simulink model "HA_sim"  (R2023b)
settings: Solver=VariableStepAuto  StartTime=0.0  StopTime=10.0  RelTol=1e-3
InitFcn:
  | HA_Parameters;
values from neighbouring files (symbols this model uses):
  g = 9.81    [HA_Parameters.m]
  J = 10.4    [HA_Parameters.m]
  l = 1.5    [HA_Parameters.m]
  L = 2    [HA_Parameters.m]
  m = 5    [HA_Parameters.m]
  M = 75    [HA_Parameters.m]
libraries: vrlib x5
settings Model: Creator=vcichella  LastModifiedBy=vcichella
settings ModelReferenceCC: EnableRefExpFcnMdlSchedulingChecks=on

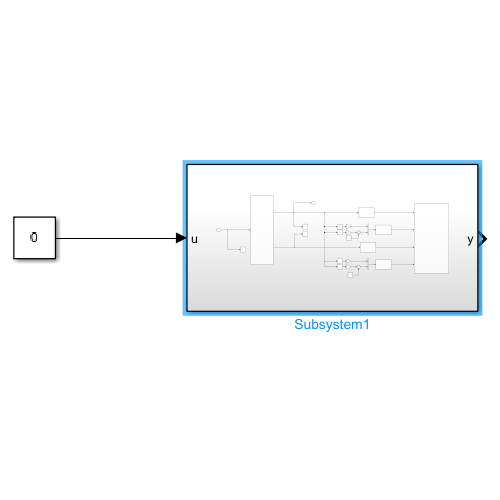
[thumbnail: Simulink's stored preview of the top-level diagram]
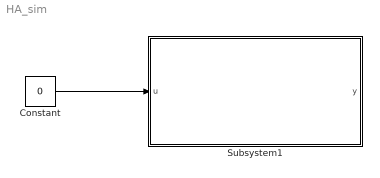
== system HA_sim ==
  Constant : Constant  Value=0
  Subsystem1 : Subsystem
  wires:
  Constant/1 -> Subsystem1/1(u)

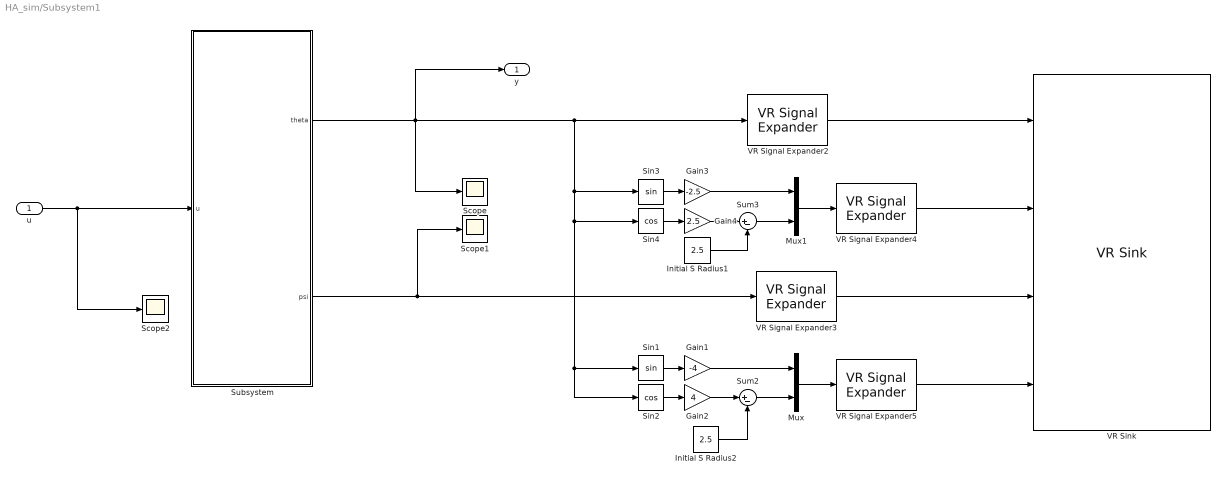
== system HA_sim/Subsystem1 ==
  u : Inport
  Gain1 : Gain  Gain=-4
  Gain2 : Gain  Gain=4
  Gain3 : Gain  Gain=-2.5
  Gain4 : Gain  Gain=2.5
  Initial S Radius1 : Constant  Value=2.5
  Initial S Radius2 : Constant  Value=2.5
  Mux : Mux  Inputs=2
  Mux1 : Mux  Inputs=2
  Scope : Scope
  Scope1 : Scope
  Scope2 : Scope
  Sin1 : Trigonometry
  Sin2 : Trigonometry  Operator=cos
  Sin3 : Trigonometry
  Sin4 : Trigonometry  Operator=cos
  Subsystem : Subsystem
  Sum2 : Sum  Inputs=|+-  InputSameDT=on  SaturateOnIntegerOverflow=on  OutDataTypeStr=Inherit: Same as first input
  Sum3 : Sum  Inputs=|+-  InputSameDT=on  SaturateOnIntegerOverflow=on  OutDataTypeStr=Inherit: Same as first input
  VR Signal Expander2 : vrlib/VR Signal Expander  outwidth=4  outidx=4
  VR Signal Expander3 : vrlib/VR Signal Expander  outwidth=4  outidx=4
  VR Signal Expander4 : vrlib/VR Signal Expander  outwidth=3  outidx=[1 2]
  VR Signal Expander5 : vrlib/VR Signal Expander  outwidth=3  outidx=[1 2]
  VR Sink : vrlib/VR Sink  InstantiateOnLoad=on  SampleTime=0.1  ViewEnable=on  RemoteChange=off  RemoteView=off  FieldsWritten=B1.rotation.4.1.1.double#B1.translation.3.1.1.double#B2.rotation.4.1.1.double#B2.translation.3.1.1.double  WorldFileName=vr_highwire.x3d  WorldDescription=vr_highwire  AutoView=on  VideoDimensions=[]  AllowVariableSize=off  FigureProperties="{'Position', 'Name', 'Viewpoint', 'CameraBound', 'CameraDirection', 'CameraPosition', 'CameraUpVector', 'ZoomFactor', 'Antialiasing', 'Headlight', 'Lighting', 'NavPanel', 'Sound', 'StatusBar', 'Stereo3D', 'Stereo3DCameraOffset', 'Stereo3DHIT', 'ToolBar', 'Textures', 'Transparency', 'Triad', 'Wireframe', 'NavZones', 'NavMode', 'NavSpeed', 'CaptureFileFormat', 'CaptureFileName', 'Record2DCompressMethod', 'Record2DCompressQuality', 'Record2D', 'Record2DFileName', 'Record2DFPS'; [2.0000000000000000e+00   9.2000000000000000e+01   5.7600000000000000e+02   3.5000000000000000e+02], 'vr_highwire', '', 'on', [0.0000000000000000e+00   0.0000000000000000e+00  -1.0000000000000000e+00], [0.0000000000000000e+00  -6.5784311294555664e-01   1.3048258590698241e+01], [0.0000000000000000e+00   1.0000000000000000e+00   0.0000000000000000e+00], [1.0000000000000000e+00], 'on', 'on', 'on', 'halfbar', 'on', 'on', 'off', [1.0000000149011612e-01], [0.0000000000000000e+00], 'on', 'on', 'on', 'none', 'off', 'off', 'fly', 'normal', 'tif', '%f_anim_%n.tif', 'auto', [7.5000000000000000e+01], 'off', '%f_anim_%n.avi', 'auto'}"
  y : Outport
  wires:
  VR Signal Expander5/1 -> VR Sink/4
  Initial S Radius2/1 -> Sum2/2
  Subsystem/2(psi) -> Scope1/1, VR Signal Expander3/1
  Sin2/1 -> Gain2/1
  u/1 -> Subsystem/1(u), Scope2/1
  Gain2/1 -> Sum2/1
  Subsystem/1(theta) -> y/1, Scope/1, Sin3/1, Sin4/1, Sin2/1, Sin1/1, VR Signal Expander2/1
  Mux/1 -> VR Signal Expander5/1
  Gain1/1 -> Mux/1
  Sin4/1 -> Gain4/1
  Sin3/1 -> Gain3/1
  Sum2/1 -> Mux/2
  Mux1/1 -> VR Signal Expander4/1
  Initial S Radius1/1 -> Sum3/2
  VR Signal Expander2/1 -> VR Sink/1
  Sin1/1 -> Gain1/1
  Gain4/1 -> Sum3/1
  Sum3/1 -> Mux1/2
  Gain3/1 -> Mux1/1
  VR Signal Expander4/1 -> VR Sink/2
  VR Signal Expander3/1 -> VR Sink/3

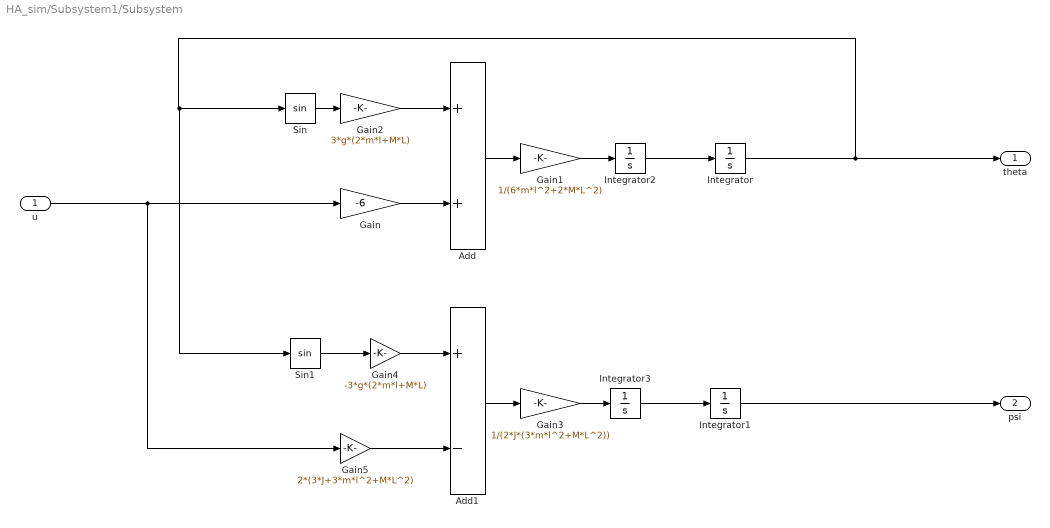
== system HA_sim/Subsystem1/Subsystem ==
  u : Inport
  Add : Sum
  Add1 : Sum  Inputs=+-
  Gain : Gain  Gain=-6
  Gain1 : Gain  Gain=1/(6*m*l^2+2*M*L^2)
  Gain2 : Gain  Gain=3*g*(2*m*l+M*L)
  Gain3 : Gain  Gain=1/(2*J*(3*m*l^2+M*L^2))
  Gain4 : Gain  Gain=-3*g*(2*m*l+M*L)
  Gain5 : Gain  Gain=2*(3*J+3*m*l^2+M*L^2)
  Integrator : Integrator  InitialCondition=pi/1000
  Integrator1 : Integrator
  Integrator2 : Integrator
  Integrator3 : Integrator
  Sin : Trigonometry
  Sin1 : Trigonometry
  theta : Outport
  psi : Outport  Port=2
  wires:
  Integrator3/1 -> Integrator1/1
  Integrator1/1 -> psi/1
  Integrator2/1 -> Integrator/1
  Integrator/1 -> Sin1/1, Sin/1, theta/1
  Add/1 -> Gain1/1
  u/1 -> Gain5/1, Gain/1
  Gain/1 -> Add/2
  Gain1/1 -> Integrator2/1
  Sin/1 -> Gain2/1
  Gain2/1 -> Add/1
  Add1/1 -> Gain3/1
  Gain3/1 -> Integrator3/1
  Sin1/1 -> Gain4/1
  Gain4/1 -> Add1/1
  Gain5/1 -> Add1/2
